simulink model "pole_placement"  (R2024b)
settings: Solver=VariableStepAuto  StartTime=0.0  StopTime=15  RelTol=1e-3
values from neighbouring files (symbols this model uses):
  A = [0 1 0 0 ... (first row only)    [calculate_k.m]
  B = [0; 0.1; 0; 0]    [calculate_k.m]
  init = [0.2; 0; 0.5; 0]    [calculate_k.m]
  K = place(A,B,p)    [calculate_k.m]
settings Model: Creator=eduar  LastModifiedBy=eduar

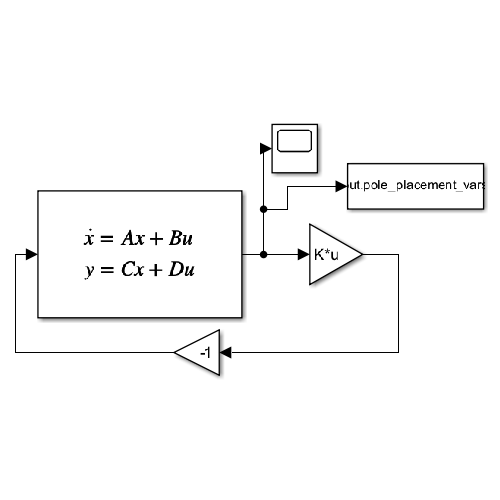
[thumbnail: Simulink's stored preview of the top-level diagram]
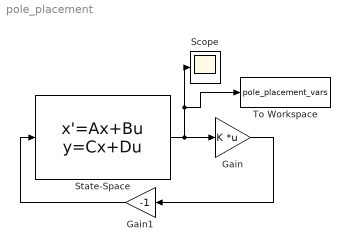
== system pole_placement ==
  Gain : Gain  Gain=K  Multiplication=Matrix(K*u)
  Gain1 : Gain  Gain=-1
  Scope : Scope
  State-Space : StateSpace  A=A  B=B  C=eye(4)  D=zeros(4,1)  InitialCondition=init
  To Workspace : ToWorkspace  VariableName=pole_placement_vars  SaveFormat=Timeseries  SampleTime=-1
  wires:
  State-Space/1 -> To Workspace/1, Scope/1, Gain/1
  Gain/1 -> Gain1/1
  Gain1/1 -> State-Space/1
